simulink model "EV_BMS_ElectroThermal_Model"  (R2026a)
settings: Solver=ode4  StopTime=SCN.t_end  FixedStep=0.25
values from neighbouring files (symbols this model uses):
  BMS = struct('I_dis_cont', 20, 'I_chg_cont', 4,      'T_warn', 45, 'T_derate', 50, 'T_cutoff', 60,      'T_chg_min', 0, 'T_chg_low', 10, 'T_chg_max', 50,      'T_cold', -20, 'V_max', 4.20, 'V_min', 2.80, 'SOC_min', 0.05,      'enable', g('bms_enable', 1))    [ev_scenario.m]
  ET = struct()    [ET_Battery_Params.m]    (also in run_Extreme_Heat_Scenarios.m = apply_cooling(ET0, S{k,7}); run_Indian_Climate_Scenarios.m = apply_cooling(ET0, S{k,6}))
  PACK = struct('Ns', 20, 'Np', 14)    [ev_scenario.m]
  SCN = struct()    [ev_scenario.m]
  VEH = struct('name', 'Electric scooter', 'm', 195,              'Cd', 0.70, 'A', 0.85, 'Crr', 0.016, 'rho', 1.18, 'kr', 1.03,              'eta_drive', 0.85, 'eta_regen', 0.50, 'P_regen_max', 2e3,              'P_trac_max', 6e3, 'v_regen_min', 5)    [ev_scenario.m]
libraries: sl_discontinuities x1
settings Model: Creator=anand  LastModifiedBy=anand

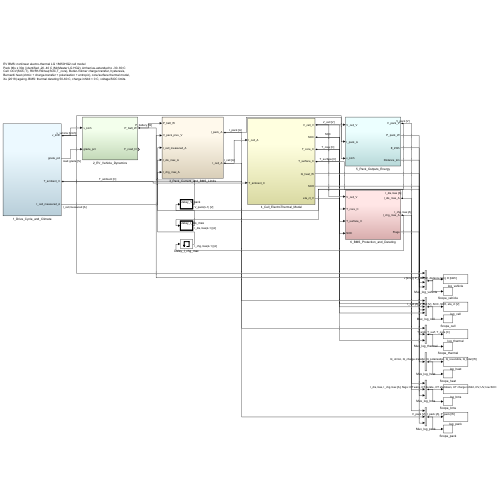
[thumbnail: Simulink's stored preview of the top-level diagram]
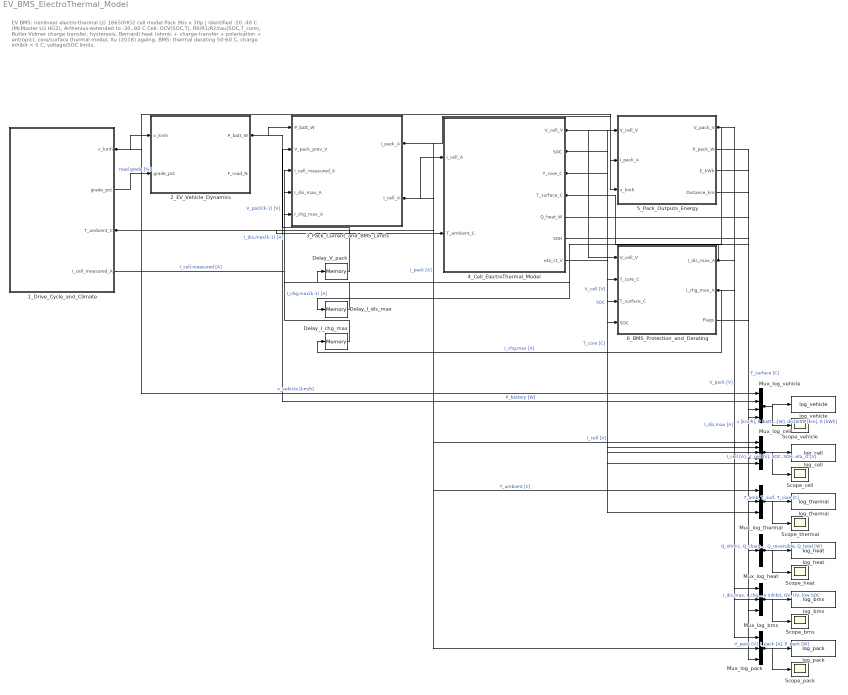
== system EV_BMS_ElectroThermal_Model ==
  note: EV BMS: nonlinear electro-thermal LG 18650HG2 cell model
      | Pack 96s x 30p | identified -20..40 C (McMaster LG HG2), Arrhenius-extended to -30..80 C
      | Cell: OCV(SOC,T), R0/R1/R2/tau(SOC,T_core), Butler-Volmer charge transfer, hysteresis,
      | Bernardi heat (ohmic + charge-transfer + polarisation + entropic), core/surface thermal model,
      | Xu (2018) ageing. BMS: thermal derating 50-60 C, charge inhibit < 0 C, voltage/SOC limits.
  1_Drive_Cycle_and_Climate : Subsystem
  2_EV_Vehicle_Dynamics : Subsystem
  3_Pack_Current_and_BMS_Limits : Subsystem
  4_Cell_ElectroThermal_Model : Subsystem
  5_Pack_Outputs_Energy : Subsystem
  6_BMS_Protection_and_Derating : Subsystem
  Delay_I_chg_max : Memory  InitialCondition=BMS.I_chg_cont*PACK.Np
  Delay_I_dis_max : Memory  InitialCondition=BMS.I_dis_cont*PACK.Np
  Delay_V_pack : Memory  InitialCondition=PACK.Ns*3.7
  Mux_log_bms : Mux  Inputs=3
  Mux_log_cell : Mux  Inputs=5
  Mux_log_heat : Mux  Inputs=1
  Mux_log_pack : Mux  Inputs=3
  Mux_log_thermal : Mux  Inputs=3
  Mux_log_vehicle : Mux
  Scope_bms : Scope
  Scope_cell : Scope
  Scope_heat : Scope
  Scope_pack : Scope
  Scope_thermal : Scope
  Scope_vehicle : Scope
  log_bms : ToWorkspace  VariableName=log_bms  SaveFormat=Timeseries  SampleTime=-1
  log_cell : ToWorkspace  VariableName=log_cell  SaveFormat=Timeseries  SampleTime=-1
  log_heat : ToWorkspace  VariableName=log_heat  SaveFormat=Timeseries  SampleTime=-1
  log_pack : ToWorkspace  VariableName=log_pack  SaveFormat=Timeseries  SampleTime=-1
  log_thermal : ToWorkspace  VariableName=log_thermal  SaveFormat=Timeseries  SampleTime=-1
  log_vehicle : ToWorkspace  VariableName=log_vehicle  SaveFormat=Timeseries  SampleTime=-1
  wires:
  1_Drive_Cycle_and_Climate/1(v_kmh) -> 2_EV_Vehicle_Dynamics/1(v_kmh), 5_Pack_Outputs_Energy/3(v_kmh), Mux_log_vehicle/1  "v_vehicle [km/h]"
  1_Drive_Cycle_and_Climate/2(grade_pct) -> 2_EV_Vehicle_Dynamics/2(grade_pct)  "road grade [%]"
  1_Drive_Cycle_and_Climate/3(T_ambient_C) -> 4_Cell_ElectroThermal_Model/2(T_ambient_C), Mux_log_thermal/1  "T_ambient [C]"
  1_Drive_Cycle_and_Climate/4(I_cell_measured_A) -> 3_Pack_Current_and_BMS_Limits/3(I_cell_measured_A)  "I_cell,measured [A]"
  2_EV_Vehicle_Dynamics/1(P_batt_W) -> 3_Pack_Current_and_BMS_Limits/1(P_batt_W), Mux_log_vehicle/2  "P_battery [W]"
  Delay_V_pack/1 -> 3_Pack_Current_and_BMS_Limits/2(V_pack_prev_V)  "V_pack(k-1) [V]"
  Delay_I_dis_max/1 -> 3_Pack_Current_and_BMS_Limits/4(I_dis_max_A)  "I_dis,max(k-1) [A]"
  Delay_I_chg_max/1 -> 3_Pack_Current_and_BMS_Limits/5(I_chg_max_A)  "I_chg,max(k-1) [A]"
  3_Pack_Current_and_BMS_Limits/2(I_cell_A) -> 4_Cell_ElectroThermal_Model/1(I_cell_A), Mux_log_cell/1  "I_cell [A]"
  3_Pack_Current_and_BMS_Limits/1(I_pack_A) -> 5_Pack_Outputs_Energy/2(I_pack_A), Mux_log_pack/2  "I_pack [A]"
  4_Cell_ElectroThermal_Model/1(V_cell_V) -> 5_Pack_Outputs_Energy/1(V_cell_V), 6_BMS_Protection_and_Derating/1(V_cell_V), Mux_log_cell/2  "V_cell [V]"
  5_Pack_Outputs_Energy/1(V_pack_V) -> Delay_V_pack/1, Mux_log_pack/1  "V_pack [V]"
  4_Cell_ElectroThermal_Model/3(T_core_C) -> 6_BMS_Protection_and_Derating/2(T_core_C), Mux_log_thermal/3  "T_core [C]"
  4_Cell_ElectroThermal_Model/4(T_surface_C) -> 6_BMS_Protection_and_Derating/3(T_surface_C), Mux_log_thermal/2  "T_surface [C]"
  4_Cell_ElectroThermal_Model/2(SOC) -> 6_BMS_Protection_and_Derating/4(SOC), Mux_log_cell/3  "SOC"
  6_BMS_Protection_and_Derating/1(I_dis_max_A) -> Delay_I_dis_max/1, Mux_log_bms/1  "I_dis,max [A]"
  6_BMS_Protection_and_Derating/2(I_chg_max_A) -> Delay_I_chg_max/1, Mux_log_bms/2  "I_chg,max [A]"
  5_Pack_Outputs_Energy/4(Distance_km) -> Mux_log_vehicle/3
  5_Pack_Outputs_Energy/3(E_kWh) -> Mux_log_vehicle/4
  Mux_log_vehicle/1 -> log_vehicle/1, Scope_vehicle/1  "v [km/h], P_batt [W], distance [km], E [kWh]"
  4_Cell_ElectroThermal_Model/6(SOH) -> Mux_log_cell/4
  4_Cell_ElectroThermal_Model/7(eta_ct_V) -> Mux_log_cell/5
  Mux_log_cell/1 -> log_cell/1, Scope_cell/1  "I_cell [A], V_cell [V], SOC, SOH, eta_ct [V]"
  Mux_log_thermal/1 -> log_thermal/1, Scope_thermal/1  "T_amb, T_surf, T_core [C]"
  4_Cell_ElectroThermal_Model/5(Q_heat_W) -> Mux_log_heat/1
  Mux_log_heat/1 -> log_heat/1, Scope_heat/1  "Q_ohmic, Q_charge-transfer, Q_polarisation, Q_reversible, Q_total [W]"
  6_BMS_Protection_and_Derating/3(Flags) -> Mux_log_bms/3
  Mux_log_bms/1 -> log_bms/1, Scope_bms/1  "I_dis,max, I_chg,max [A], flags: OT warn, OT derate, OT shutdown, UT charge inhibit, OV, UV, low SOC"
  5_Pack_Outputs_Energy/2(P_pack_W) -> Mux_log_pack/3
  Mux_log_pack/1 -> log_pack/1, Scope_pack/1  "V_pack [V], I_pack [A], P_pack [W]"

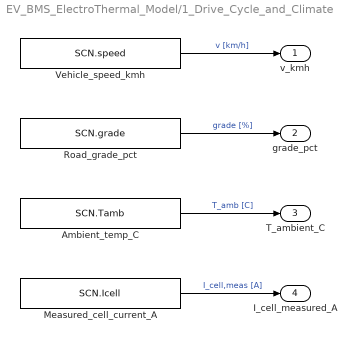
== system EV_BMS_ElectroThermal_Model/1_Drive_Cycle_and_Climate ==
  Ambient_temp_C : FromWorkspace  VariableName=SCN.Tamb  OutputAfterFinalValue=Holding final value
  Measured_cell_current_A : FromWorkspace  VariableName=SCN.Icell  Interpolate=off  OutputAfterFinalValue=Holding final value
  Road_grade_pct : FromWorkspace  VariableName=SCN.grade  OutputAfterFinalValue=Holding final value
  Vehicle_speed_kmh : FromWorkspace  VariableName=SCN.speed  OutputAfterFinalValue=Holding final value
  v_kmh : Outport
  grade_pct : Outport  Port=2
  T_ambient_C : Outport  Port=3
  I_cell_measured_A : Outport  Port=4
  wires:
  Vehicle_speed_kmh/1 -> v_kmh/1  "v [km/h]"
  Road_grade_pct/1 -> grade_pct/1  "grade [%]"
  Ambient_temp_C/1 -> T_ambient_C/1  "T_amb [C]"
  Measured_cell_current_A/1 -> I_cell_measured_A/1  "I_cell,meas [A]"

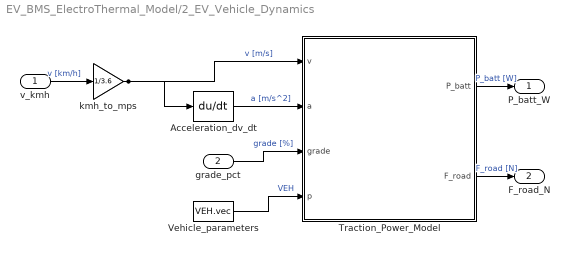
== system EV_BMS_ElectroThermal_Model/2_EV_Vehicle_Dynamics ==
  v_kmh : Inport
  grade_pct : Inport  Port=2
  Acceleration_dv_dt : Derivative
  Traction_Power_Model : MATLAB Function  TreatAsAtomicUnit=on
  Vehicle_parameters : Constant  Value=VEH.vec
  kmh_to_mps : Gain  Gain=1/3.6
  P_batt_W : Outport
  F_road_N : Outport  Port=2
  wires:
  v_kmh/1 -> kmh_to_mps/1  "v [km/h]"
  Traction_Power_Model/2(F_road) -> F_road_N/1  "F_road [N]"
  kmh_to_mps/1 -> Traction_Power_Model/1(v), Acceleration_dv_dt/1  "v [m/s]"
  Vehicle_parameters/1 -> Traction_Power_Model/4(p)  "VEH"
  Acceleration_dv_dt/1 -> Traction_Power_Model/2(a)  "a [m/s^2]"
  grade_pct/1 -> Traction_Power_Model/3(grade)  "grade [%]"
  Traction_Power_Model/1(P_batt) -> P_batt_W/1  "P_batt [W]"

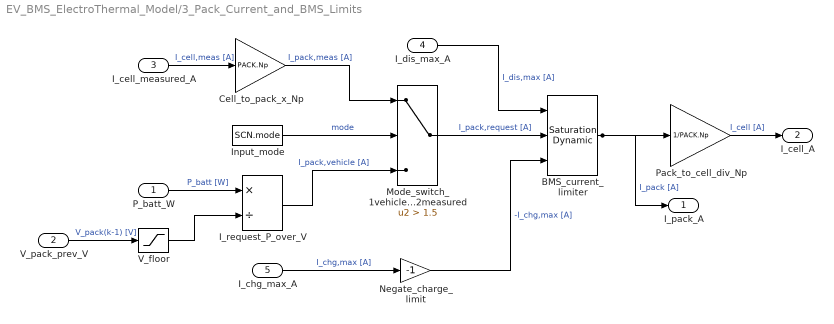
== system EV_BMS_ElectroThermal_Model/3_Pack_Current_and_BMS_Limits ==
  P_batt_W : Inport
  V_pack_prev_V : Inport  Port=2
  I_cell_measured_A : Inport  Port=3
  I_dis_max_A : Inport  Port=4
  I_chg_max_A : Inport  Port=5
  BMS_current_limiter : sl_discontinuities/Saturation Dynamic  OutMin=[]  OutMax=[]  OutDataTypeStr=Inherit: Same as second input  OutDataType=fixdt(1, 16)  OutScaling=2^-10  DoSatur=off
      settings: LibrarySourceBlock=|
      | simulink/Discontinuities/Saturation
      | Dynamic
  Cell_to_pack_x_Np : Gain  Gain=PACK.Np
  I_request_P_over_V : Product  Inputs=*/
  Input_mode : Constant  Value=SCN.mode
  Mode_switch_1vehicle_2measured : Switch  Criteria=u2 > Threshold  Threshold=1.5  SaturateOnIntegerOverflow=off  InputSameDT=off
  Negate_charge_limit : Gain  Gain=-1
  Pack_to_cell_div_Np : Gain  Gain=1/PACK.Np
  V_floor : Saturate  UpperLimit=inf  LowerLimit=1
  I_pack_A : Outport
  I_cell_A : Outport  Port=2
  wires:
  I_chg_max_A/1 -> Negate_charge_limit/1  "I_chg,max [A]"
  P_batt_W/1 -> I_request_P_over_V/1  "P_batt [W]"
  V_floor/1 -> I_request_P_over_V/2
  I_request_P_over_V/1 -> Mode_switch_1vehicle_2measured/3  "I_pack,vehicle [A]"
  Input_mode/1 -> Mode_switch_1vehicle_2measured/2  "mode"
  Cell_to_pack_x_Np/1 -> Mode_switch_1vehicle_2measured/1  "I_pack,meas [A]"
  I_cell_measured_A/1 -> Cell_to_pack_x_Np/1  "I_cell,meas [A]"
  V_pack_prev_V/1 -> V_floor/1  "V_pack(k-1) [V]"
  I_dis_max_A/1 -> BMS_current_limiter/1  "I_dis,max [A]"
  Mode_switch_1vehicle_2measured/1 -> BMS_current_limiter/2  "I_pack,request [A]"
  Negate_charge_limit/1 -> BMS_current_limiter/3  "-I_chg,max [A]"
  BMS_current_limiter/1 -> I_pack_A/1, Pack_to_cell_div_Np/1  "I_pack [A]"
  Pack_to_cell_div_Np/1 -> I_cell_A/1  "I_cell [A]"

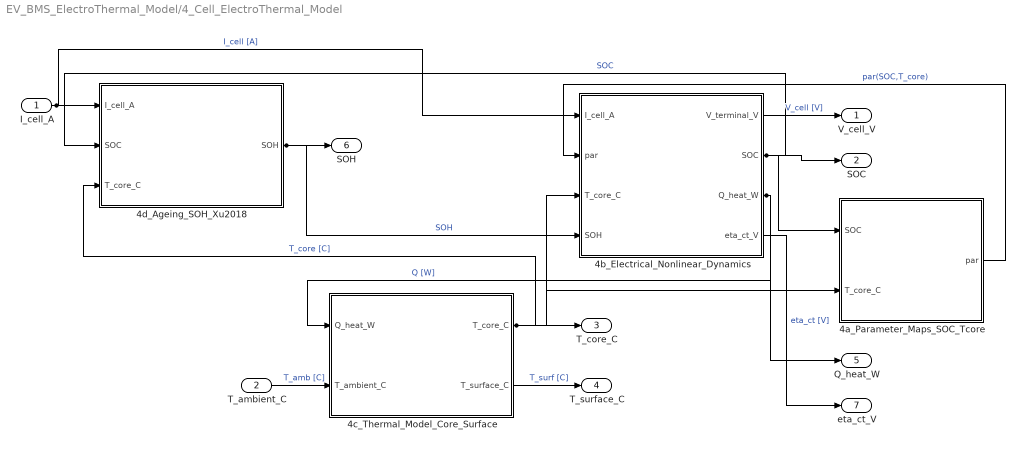
== system EV_BMS_ElectroThermal_Model/4_Cell_ElectroThermal_Model ==
  I_cell_A : Inport
  T_ambient_C : Inport  Port=2
  4a_Parameter_Maps_SOC_Tcore : Subsystem
  4b_Electrical_Nonlinear_Dynamics : Subsystem
  4c_Thermal_Model_Core_Surface : Subsystem
  4d_Ageing_SOH_Xu2018 : Subsystem
  V_cell_V : Outport
  SOC : Outport  Port=2
  T_core_C : Outport  Port=3
  T_surface_C : Outport  Port=4
  Q_heat_W : Outport  Port=5
  SOH : Outport  Port=6
  eta_ct_V : Outport  Port=7
  wires:
  4b_Electrical_Nonlinear_Dynamics/3(Q_heat_W) -> 4c_Thermal_Model_Core_Surface/1(Q_heat_W), Q_heat_W/1  "Q [W]"
  4b_Electrical_Nonlinear_Dynamics/1(V_terminal_V) -> V_cell_V/1  "V_cell [V]"
  T_ambient_C/1 -> 4c_Thermal_Model_Core_Surface/2(T_ambient_C)  "T_amb [C]"
  I_cell_A/1 -> 4b_Electrical_Nonlinear_Dynamics/1(I_cell_A), 4d_Ageing_SOH_Xu2018/1(I_cell_A)  "I_cell [A]"
  4d_Ageing_SOH_Xu2018/1(SOH) -> 4b_Electrical_Nonlinear_Dynamics/4(SOH), SOH/1  "SOH"
  4c_Thermal_Model_Core_Surface/1(T_core_C) -> 4d_Ageing_SOH_Xu2018/3(T_core_C), 4a_Parameter_Maps_SOC_Tcore/2(T_core_C), 4b_Electrical_Nonlinear_Dynamics/3(T_core_C), T_core_C/1  "T_core [C]"
  4c_Thermal_Model_Core_Surface/2(T_surface_C) -> T_surface_C/1  "T_surf [C]"
  4b_Electrical_Nonlinear_Dynamics/2(SOC) -> 4d_Ageing_SOH_Xu2018/2(SOC), 4a_Parameter_Maps_SOC_Tcore/1(SOC), SOC/1  "SOC"
  4b_Electrical_Nonlinear_Dynamics/4(eta_ct_V) -> eta_ct_V/1  "eta_ct [V]"
  4a_Parameter_Maps_SOC_Tcore/1(par) -> 4b_Electrical_Nonlinear_Dynamics/2(par)  "par(SOC,T_core)"

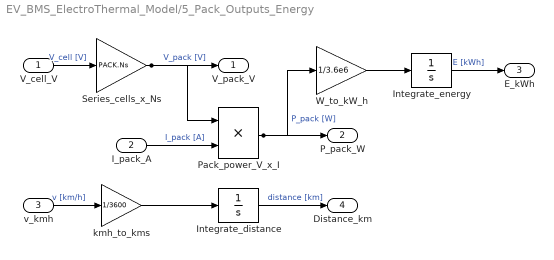
== system EV_BMS_ElectroThermal_Model/5_Pack_Outputs_Energy ==
  V_cell_V : Inport
  I_pack_A : Inport  Port=2
  v_kmh : Inport  Port=3
  Integrate_distance : Integrator
  Integrate_energy : Integrator
  Pack_power_V_x_I : Product
  Series_cells_x_Ns : Gain  Gain=PACK.Ns
  W_to_kW_h : Gain  Gain=1/3.6e6
  kmh_to_kms : Gain  Gain=1/3600
  V_pack_V : Outport
  P_pack_W : Outport  Port=2
  E_kWh : Outport  Port=3
  Distance_km : Outport  Port=4
  wires:
  Integrate_distance/1 -> Distance_km/1  "distance [km]"
  Pack_power_V_x_I/1 -> P_pack_W/1, W_to_kW_h/1  "P_pack [W]"
  Series_cells_x_Ns/1 -> V_pack_V/1, Pack_power_V_x_I/1  "V_pack [V]"
  v_kmh/1 -> kmh_to_kms/1  "v [km/h]"
  Integrate_energy/1 -> E_kWh/1  "E [kWh]"
  V_cell_V/1 -> Series_cells_x_Ns/1  "V_cell [V]"
  W_to_kW_h/1 -> Integrate_energy/1
  I_pack_A/1 -> Pack_power_V_x_I/2  "I_pack [A]"
  kmh_to_kms/1 -> Integrate_distance/1

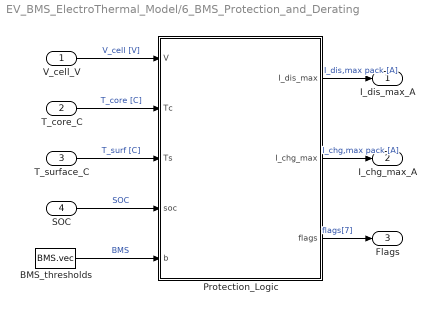
== system EV_BMS_ElectroThermal_Model/6_BMS_Protection_and_Derating ==
  V_cell_V : Inport
  T_core_C : Inport  Port=2
  T_surface_C : Inport  Port=3
  SOC : Inport  Port=4
  BMS_thresholds : Constant  Value=BMS.vec
  Protection_Logic : MATLAB Function  TreatAsAtomicUnit=on
  I_dis_max_A : Outport
  I_chg_max_A : Outport  Port=2
  Flags : Outport  Port=3
  wires:
  V_cell_V/1 -> Protection_Logic/1(V)  "V_cell [V]"
  Protection_Logic/2(I_chg_max) -> I_chg_max_A/1  "I_chg,max pack [A]"
  SOC/1 -> Protection_Logic/4(soc)  "SOC"
  T_core_C/1 -> Protection_Logic/2(Tc)  "T_core [C]"
  Protection_Logic/3(flags) -> Flags/1  "flags[7]"
  Protection_Logic/1(I_dis_max) -> I_dis_max_A/1  "I_dis,max pack [A]"
  BMS_thresholds/1 -> Protection_Logic/5(b)  "BMS"
  T_surface_C/1 -> Protection_Logic/3(Ts)  "T_surf [C]"

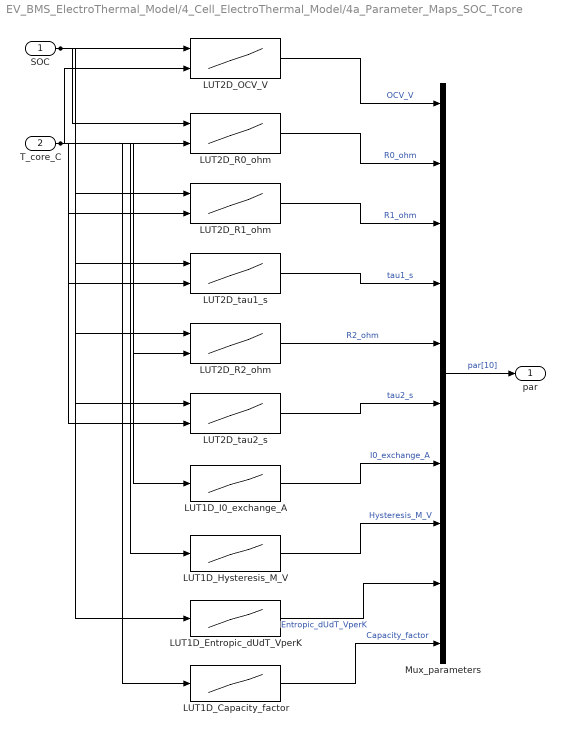
== system EV_BMS_ElectroThermal_Model/4_Cell_ElectroThermal_Model/4a_Parameter_Maps_SOC_Tcore ==
  SOC : Inport
  T_core_C : Inport  Port=2
  LUT1D_Capacity_factor : Lookup_n-D  NumberOfTableDimensions=1  BreakpointsForDimension1=ET.T_bp  Table=ET.cap_factor  ExtrapMethod=Clip  InternalRulePriority=Speed  RndMeth=Simplest
  LUT1D_Entropic_dUdT_VperK : Lookup_n-D  NumberOfTableDimensions=1  BreakpointsForDimension1=ET.soc_bp  Table=ET.dUdT  ExtrapMethod=Clip  InternalRulePriority=Speed  RndMeth=Simplest
  LUT1D_Hysteresis_M_V : Lookup_n-D  NumberOfTableDimensions=1  BreakpointsForDimension1=ET.T_bp  Table=ET.hyst_M  ExtrapMethod=Clip  InternalRulePriority=Speed  RndMeth=Simplest
  LUT1D_I0_exchange_A : Lookup_n-D  NumberOfTableDimensions=1  BreakpointsForDimension1=ET.T_bp  Table=ET.I0  ExtrapMethod=Clip  InternalRulePriority=Speed  RndMeth=Simplest
  LUT2D_OCV_V : Lookup_n-D  BreakpointsForDimension1=ET.soc_bp  BreakpointsForDimension2=ET.T_bp  Table=ET.OCV  ExtrapMethod=Clip  InternalRulePriority=Speed  RndMeth=Simplest
      settings: InputPortMap=u0,u1
  LUT2D_R0_ohm : Lookup_n-D  BreakpointsForDimension1=ET.soc_bp  BreakpointsForDimension2=ET.T_bp  Table=ET.R0  ExtrapMethod=Clip  InternalRulePriority=Speed  RndMeth=Simplest
      settings: InputPortMap=u0,u1
  LUT2D_R1_ohm : Lookup_n-D  BreakpointsForDimension1=ET.soc_bp  BreakpointsForDimension2=ET.T_bp  Table=ET.R1  ExtrapMethod=Clip  InternalRulePriority=Speed  RndMeth=Simplest
      settings: InputPortMap=u0,u1
  LUT2D_R2_ohm : Lookup_n-D  BreakpointsForDimension1=ET.soc_bp  BreakpointsForDimension2=ET.T_bp  Table=ET.R2  ExtrapMethod=Clip  InternalRulePriority=Speed  RndMeth=Simplest
      settings: InputPortMap=u0,u1
  LUT2D_tau1_s : Lookup_n-D  BreakpointsForDimension1=ET.soc_bp  BreakpointsForDimension2=ET.T_bp  Table=ET.tau1  ExtrapMethod=Clip  InternalRulePriority=Speed  RndMeth=Simplest
      settings: InputPortMap=u0,u1
  LUT2D_tau2_s : Lookup_n-D  BreakpointsForDimension1=ET.soc_bp  BreakpointsForDimension2=ET.T_bp  Table=ET.tau2  ExtrapMethod=Clip  InternalRulePriority=Speed  RndMeth=Simplest
      settings: InputPortMap=u0,u1
  Mux_parameters : Mux  Inputs=10
  par : Outport
  wires:
  T_core_C/1 -> LUT2D_OCV_V/2, LUT2D_R1_ohm/2, LUT2D_R2_ohm/2, LUT2D_tau1_s/2, LUT1D_I0_exchange_A/1, LUT1D_Hysteresis_M_V/1, LUT2D_tau2_s/2, LUT2D_R0_ohm/2, LUT1D_Capacity_factor/1
  SOC/1 -> LUT2D_tau1_s/1, LUT2D_tau2_s/1, LUT2D_R2_ohm/1, LUT2D_R0_ohm/1, LUT2D_OCV_V/1, LUT1D_Entropic_dUdT_VperK/1, LUT2D_R1_ohm/1
  LUT2D_R0_ohm/1 -> Mux_parameters/2  "R0_ohm"
  LUT2D_tau1_s/1 -> Mux_parameters/4  "tau1_s"
  LUT2D_OCV_V/1 -> Mux_parameters/1  "OCV_V"
  LUT2D_R1_ohm/1 -> Mux_parameters/3  "R1_ohm"
  LUT2D_tau2_s/1 -> Mux_parameters/6  "tau2_s"
  LUT1D_I0_exchange_A/1 -> Mux_parameters/7  "I0_exchange_A"
  LUT2D_R2_ohm/1 -> Mux_parameters/5  "R2_ohm"
  LUT1D_Hysteresis_M_V/1 -> Mux_parameters/8  "Hysteresis_M_V"
  LUT1D_Entropic_dUdT_VperK/1 -> Mux_parameters/9  "Entropic_dUdT_VperK"
  LUT1D_Capacity_factor/1 -> Mux_parameters/10  "Capacity_factor"
  Mux_parameters/1 -> par/1  "par[10]"

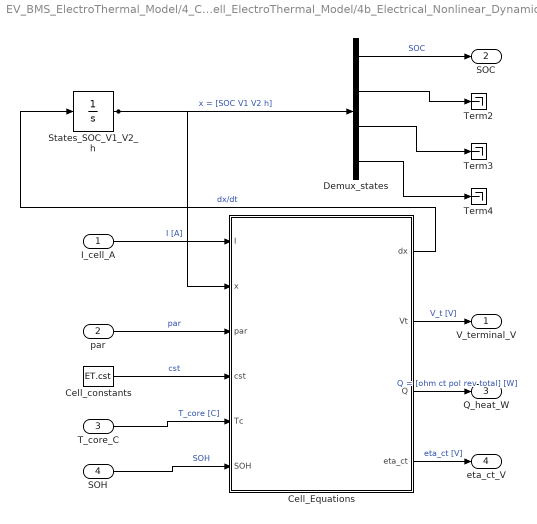
== system EV_BMS_ElectroThermal_Model/4_Cell_ElectroThermal_Model/4b_Electrical_Nonlinear_Dynamics ==
  I_cell_A : Inport
  par : Inport  Port=2
  T_core_C : Inport  Port=3
  SOH : Inport  Port=4
  Cell_Equations : MATLAB Function  TreatAsAtomicUnit=on
  Cell_constants : Constant  Value=ET.cst
  Demux_states : Demux
  States_SOC_V1_V2_h : Integrator  InitialCondition=[SCN.soc0; 0; 0; 0]
  Term2 : Terminator
  Term3 : Terminator
  Term4 : Terminator
  V_terminal_V : Outport
  SOC : Outport  Port=2
  Q_heat_W : Outport  Port=3
  eta_ct_V : Outport  Port=4
  wires:
  Cell_Equations/4(eta_ct) -> eta_ct_V/1  "eta_ct [V]"
  States_SOC_V1_V2_h/1 -> Cell_Equations/2(x), Demux_states/1  "x = [SOC V1 V2 h]"
  I_cell_A/1 -> Cell_Equations/1(I)  "I [A]"
  Demux_states/2 -> Term2/1
  T_core_C/1 -> Cell_Equations/5(Tc)  "T_core [C]"
  par/1 -> Cell_Equations/3(par)  "par"
  SOH/1 -> Cell_Equations/6(SOH)  "SOH"
  Cell_constants/1 -> Cell_Equations/4(cst)  "cst"
  Demux_states/1 -> SOC/1  "SOC"
  Demux_states/3 -> Term3/1
  Demux_states/4 -> Term4/1
  Cell_Equations/1(dx) -> States_SOC_V1_V2_h/1  "dx/dt"
  Cell_Equations/2(Vt) -> V_terminal_V/1  "V_t [V]"
  Cell_Equations/3(Q) -> Q_heat_W/1  "Q = [ohm ct pol rev total] [W]"

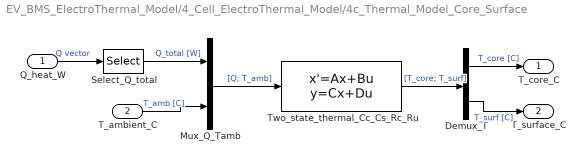
== system EV_BMS_ElectroThermal_Model/4_Cell_ElectroThermal_Model/4c_Thermal_Model_Core_Surface ==
  Q_heat_W : Inport
  T_ambient_C : Inport  Port=2
  Demux_T : Demux  Outputs=2
  Mux_Q_Tamb : Mux  Inputs=2
  Select_Q_total : Selector  InputPortWidth=5  IndexOptions=Index vector (dialog)  Indices=5  OutputSizes=1
  Two_state_thermal_Cc_Cs_Rc_Ru : StateSpace  A=ET.A_th  B=ET.B_th  C=eye(2)  D=zeros(2)  InitialCondition=[SCN.T0; SCN.T0]
  T_core_C : Outport
  T_surface_C : Outport  Port=2
  wires:
  Two_state_thermal_Cc_Cs_Rc_Ru/1 -> Demux_T/1  "[T_core; T_surf]"
  Mux_Q_Tamb/1 -> Two_state_thermal_Cc_Cs_Rc_Ru/1  "[Q; T_amb]"
  Select_Q_total/1 -> Mux_Q_Tamb/1  "Q_total [W]"
  Q_heat_W/1 -> Select_Q_total/1  "Q vector"
  T_ambient_C/1 -> Mux_Q_Tamb/2  "T_amb [C]"
  Demux_T/1 -> T_core_C/1  "T_core [C]"
  Demux_T/2 -> T_surface_C/1  "T_surf [C]"

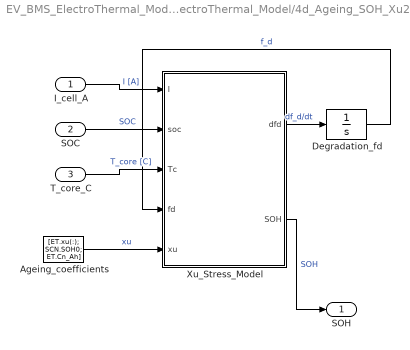
== system EV_BMS_ElectroThermal_Model/4_Cell_ElectroThermal_Model/4d_Ageing_SOH_Xu2018 ==
  I_cell_A : Inport
  SOC : Inport  Port=2
  T_core_C : Inport  Port=3
  Ageing_coefficients : Constant  Value=[ET.xu(:); SCN.SOH0; ET.Cn_Ah]
  Degradation_fd : Integrator
  Xu_Stress_Model : MATLAB Function  TreatAsAtomicUnit=on
  SOH : Outport
  wires:
  Degradation_fd/1 -> Xu_Stress_Model/4(fd)  "f_d"
  Xu_Stress_Model/1(dfd) -> Degradation_fd/1  "df_d/dt"
  T_core_C/1 -> Xu_Stress_Model/3(Tc)  "T_core [C]"
  I_cell_A/1 -> Xu_Stress_Model/1(I)  "I [A]"
  Ageing_coefficients/1 -> Xu_Stress_Model/5(xu)  "xu"
  SOC/1 -> Xu_Stress_Model/2(soc)  "SOC"
  Xu_Stress_Model/2(SOH) -> SOH/1  "SOH"

== matlab function EV_BMS_ElectroThermal_Model/4_Cell_ElectroThermal_Model/4b_Electrical_Nonlinear_Dynamics/Cell_Equations ==
  data: I input; dx output; x input; par input; cst input; Tc input; SOH input; Vt output; Q output; eta_ct output
function [dx, Vt, Q, eta_ct] = Cell_Equations(I, x, par, cst, Tc, SOH)
%#codegen
% Nonlinear electro-thermal cell, I > 0 discharge. x = [SOC; V1; V2; h]
% par = [OCV R0 R1 tau1 R2 tau2 I0 M dUdT capf] at (SOC, T_core)
% cst = [Cn_Ah eta_chg gamma k_R]
soc = x(1); v1 = x(2); v2 = x(3); h = x(4);
Cn = cst(1); eta_chg = cst(2); gam = cst(3); kR = cst(4);
SOH = max(SOH, 0.5);
g = 1 + kR*(1 - SOH);                   % resistance growth with ageing
OCV = par(1); R0 = g*par(2); R1 = g*par(3); tau1 = max(par(4), 1e-3);
R2 = g*par(5); tau2 = max(par(6), 1e-3); I0 = max(par(7), 1e-3)/g;
M = par(8); dUdT = par(9); capf = par(10);
TK = Tc + 273.15;
% Butler-Volmer charge-transfer overpotential (theoretical Tafel slope)
eta_ct = 2*8.314462618*TK/96485.33212*asinh(I/(2*I0));
if I >= 0
    eta = 1;
else
    eta = eta_chg;
end
dsoc = -eta*I/(3600*Cn*capf*SOH);
dv1 = (R1*I - v1)/tau1;                 % fast polarisation
dv2 = (R2*I - v2)/tau2;                 % diffusion polarisation
dh  = -gam*abs(dsoc)*(h + sign(I));     % one-state hysteresis (Plett)
dx = [dsoc; dv1; dv2; dh];
Vt = OCV + M*h - I*R0 - eta_ct - v1 - v2;
% Bernardi heat generation [W]: Q = I*(OCV - Vt) - I*T*dU/dT, split by source
Q_ohm = I^2*R0;
Q_ct  = I*eta_ct;
Q_pol = I*(v1 + v2);                   % Bernardi: current x polarisation
Q_rev = -I*TK*dUdT;
Q = [Q_ohm; Q_ct; Q_pol; Q_rev; Q_ohm + Q_ct + Q_pol + Q_rev];
end

== matlab function EV_BMS_ElectroThermal_Model/2_EV_Vehicle_Dynamics/Traction_Power_Model ==
  data: v input; P_batt output; a input; grade input; p input; F_road output
function [P_batt, F_road] = Traction_Power_Model(v, a, grade, p)
%#codegen
% Longitudinal EV dynamics. v [m/s], a [m/s^2], grade [%], p = VEH.vec
% p = [m Cd A Crr rho kr eta_drive eta_regen P_regen_max P_aux v_regen_min P_trac_max]
m = p(1); Cd = p(2); A = p(3); Crr = p(4); rho = p(5); kr = p(6);
eta_d = p(7); eta_r = p(8); Preg_max = p(9); P_aux = p(10);
v_reg_min = p(11)/3.6; Ptr_max = p(12);
th = atan(grade/100);
F_aero  = 0.5*rho*Cd*A*v^2;
F_roll  = m*9.81*Crr*cos(th)*(v > 0.1);
F_grade = m*9.81*sin(th);
F_inert = kr*m*a;
F_road = F_aero + F_roll + F_grade + F_inert;
P_wheel = F_road*v;
if P_wheel >= 0
    P_mot = min(P_wheel, Ptr_max)/eta_d;          % traction
elseif v > v_reg_min
    P_mot = max(P_wheel*eta_r, -Preg_max);        % regenerative braking
else
    P_mot = 0;                                    % friction brakes only
end
P_batt = P_mot + P_aux;
end

== matlab function EV_BMS_ElectroThermal_Model/4_Cell_ElectroThermal_Model/4d_Ageing_SOH_Xu2018/Xu_Stress_Model ==
  data: I input; dfd output; soc input; Tc input; fd input; xu input; SOH output
function [dfd, SOH] = Xu_Stress_Model(I, soc, Tc, fd, xu)
%#codegen
% Semi-empirical degradation, Xu et al., IEEE Trans. Smart Grid 9(2), 2018.
% xu = [a_sei b_sei k_d1 k_d2 k_d3 k_s s_ref k_T T_ref k_t T_min DoD_ref SOH0 Cn]
a = xu(1); b = xu(2); kd1 = xu(3); kd2 = xu(4); kd3 = xu(5);
ks = xu(6); sref = xu(7); kT = xu(8); Tref = xu(9) + 273.15; kt = xu(10);
Tmin = xu(11); DoD = xu(12); SOH0 = xu(13); Cn = xu(14);
T = max(Tc, Tmin) + 273.15;             % law valid above 15 C (paper)
S_T = exp(kT*(T - Tref)*Tref/T);
S_s = exp(ks*(soc - sref));
S_d = 1/(kd1*DoD^kd2 + kd3);            % stress of one cycle of depth DoD
cyc_rate = abs(I)/(2*3600*Cn)/DoD;      % cycles of depth DoD per second
dfd = (kt + cyc_rate*S_d)*S_s*S_T;      % calendar + cycling
L = 1 - a*exp(-b*fd) - (1 - a)*exp(-fd);
SOH = SOH0*(1 - L);
end

== matlab function EV_BMS_ElectroThermal_Model/6_BMS_Protection_and_Derating/Protection_Logic ==
  data: V input; I_dis_max output; Tc input; Ts input; soc input; b input; I_chg_max output; flags output
function [I_dis_max, I_chg_max, flags] = Protection_Logic(V, Tc, Ts, soc, b)
%#codegen
% b = [I_dis I_chg T_warn T_derate T_cutoff T_chg_min T_chg_low T_chg_max
%      T_cold V_max V_min SOC_min Np enable]
Idis = b(1); Ichg = b(2); Tw = b(3); Td = b(4); Tcut = b(5);
Tcmin = b(6); Tclow = b(7); Tcmax = b(8); Tcold = b(9);
Vmax = b(10); Vmin = b(11); SOCmin = b(12); Np = b(13); en = b(14);
T = max(Tc, Ts);                        % hottest node (core estimate)
% discharge derating: full below T_derate, linear to zero at T_cutoff
fd = min(max((Tcut - T)/(Tcut - Td), 0), 1);
if T < Tcold, fd = 0.25*fd; end         % extreme cold: limit power
% charge window: none below T_chg_min (Li plating), half up to T_chg_low
if T < Tcmin
    fc = 0;
elseif T < Tclow
    fc = 0.5;
else
    fc = min(max((Tcmax - T)/(Tcmax - Td + 1e-6), 0), 1);
end
OV = double(V >= Vmax); UV = double(V <= Vmin); LS = double(soc <= SOCmin);
if OV > 0, fc = 0; end
if UV > 0 || LS > 0, fd = 0; end
flags = [double(T >= Tw); double(T >= Td); double(T >= Tcut); ...
         double(T < Tcmin); OV; UV; LS];
if en > 0
    I_dis_max = fd*Idis*Np; I_chg_max = fc*Ichg*Np;
else
    I_dis_max = 1e6; I_chg_max = 1e6;    % protection disabled (validation runs)
end
end
